simulink model "DP_STD_MDL_DCAC_3ph_2level_gridconn"  (R2024b)
settings: Solver=VariableStepAuto  StartTime=0.0  StopTime=6  RelTol=1e-3
libraries: spsSeriesRLCBranchLib x18, spsSecondOrderFilterLib x7, spsVoltageMeasurementLib x7, spsControlledVoltageSourceLib x4, spsMosfetLib x4, spsCurrentMeasurementLib x3, simulink x2, gmp_sil_core_pack x1, gmp_peripheral_utilities x1, spsdq0toabcLib x1, sps_lib x1
(part 2 of 2)

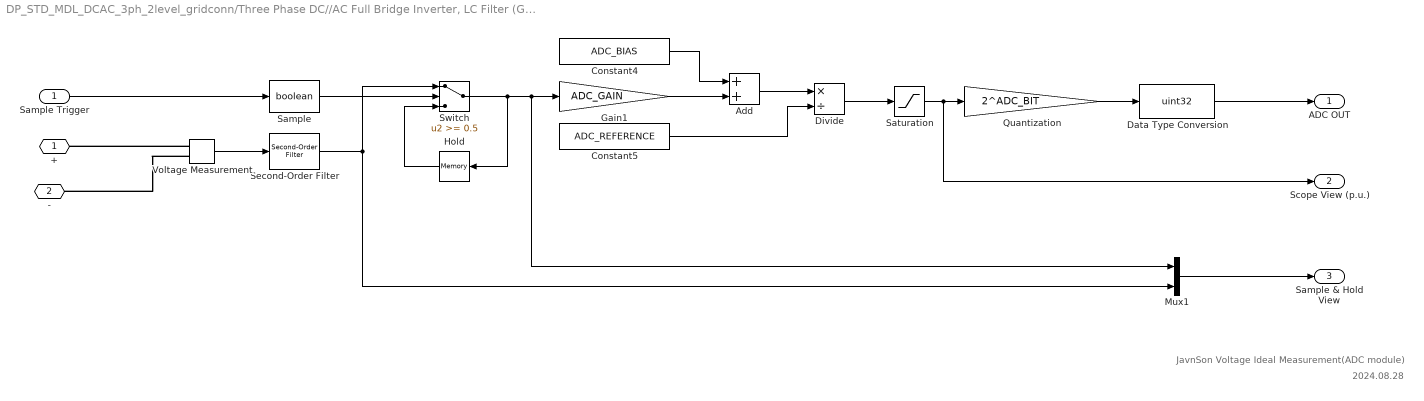
== system DP_STD_MDL_DCAC_3ph_2level_gridconn/Three Phase DC//AC Full Bridge Inverter, LC Filter (GMP STD MDL)/Capactor Voltage Uab Measurement Module1 ==
  note: 2024.08.28
  note: JavnSon Voltage Ideal Measurement(ADC module)
  Sample Trigger : Inport
  Add : Sum
  Constant4 : Constant  Value=ADC_BIAS
  Constant5 : Constant  Value=ADC_REFERENCE
  Data Type Conversion : DataTypeConversion  OutDataTypeStr=uint32  ConvertRealWorld=Stored Integer (SI)  SaturateOnIntegerOverflow=off  RndMeth=Floor
  Divide : Product  Inputs=*/
  Gain1 : Gain  Gain=ADC_GAIN
  Hold : Memory  InitialCondition=ADC_INIT  LinearizeAsDelay=on
  Mux1 : Mux  Inputs=2
  Quantization : Gain  Gain=2^ADC_BIT
  Sample : DataTypeConversion  OutDataTypeStr=boolean  SaturateOnIntegerOverflow=off  RndMeth=Floor
  Saturation : Saturate  UpperLimit=1  LowerLimit=0
  Second-Order Filter : spsSecondOrderFilterLib/Second-Order Filter  FilterType=Lowpass  Fo=cut_frequency  Zeta=0.707  Ts=0  Initialize=off  Vac_Init="[0,  0,  60]"  Vdc_Init=0  PlotResponse=off  FreqRange=[0, 500, 1]
  Switch : Switch  Threshold=0.5
  Voltage Measurement : spsVoltageMeasurementLib/Voltage Measurement  PhasorSimulation=off  OutputType=Complex  PSBequivalent=0
  + : PMIOPort  Side=Left
  - : PMIOPort  Port=2  Side=Left
  ADC OUT : Outport
  Scope View (p.u.) : Outport  Port=2
  Sample & Hold View : Outport  Port=3
  wires:
  Sample/1 -> Switch/2
  Add/1 -> Divide/1
  Constant5/1 -> Divide/2
  Quantization/1 -> Data Type Conversion/1
  Mux1/1 -> Sample & Hold View/1
  Data Type Conversion/1 -> ADC OUT/1
  Sample Trigger/1 -> Sample/1
  Gain1/1 -> Add/2
  Constant4/1 -> Add/1
  Saturation/1 -> Quantization/1, Scope View (p.u.)/1
  Voltage Measurement/1 -> Second-Order Filter/1
  Divide/1 -> Saturation/1
  Switch/1 -> Gain1/1, Mux1/1, Hold/1
  Hold/1 -> Switch/3
  Second-Order Filter/1 -> Switch/1, Mux1/2
  connections:
  Voltage Measurement/LConn2 -- -/RConn1
  Voltage Measurement/LConn1 -- +/RConn1

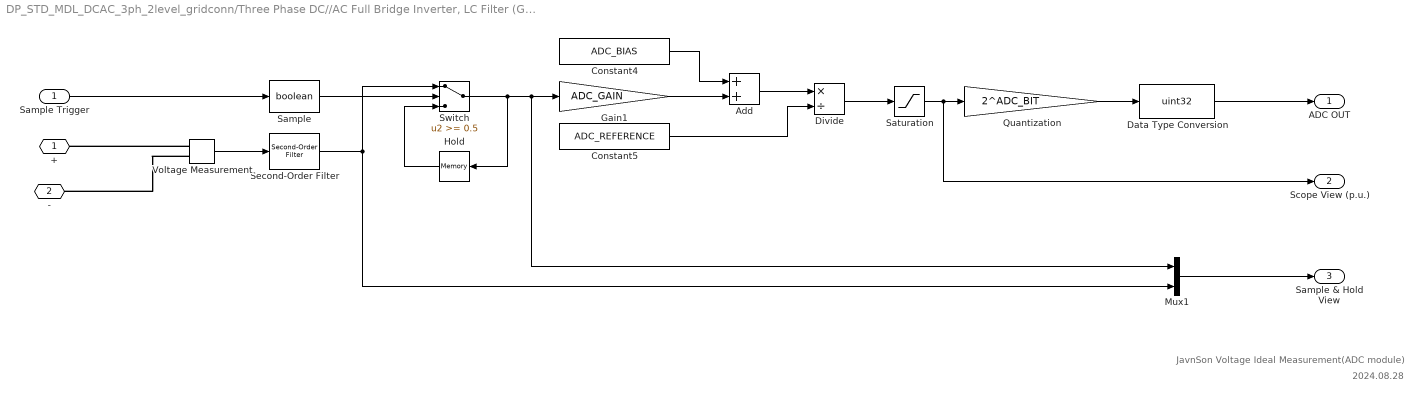
== system DP_STD_MDL_DCAC_3ph_2level_gridconn/Three Phase DC//AC Full Bridge Inverter, LC Filter (GMP STD MDL)/Capactor Voltage Ubc Measurement Module5 ==
  note: JavnSon Voltage Ideal Measurement(ADC module)
  note: 2024.08.28
  Sample Trigger : Inport
  Add : Sum
  Constant4 : Constant  Value=ADC_BIAS
  Constant5 : Constant  Value=ADC_REFERENCE
  Data Type Conversion : DataTypeConversion  OutDataTypeStr=uint32  ConvertRealWorld=Stored Integer (SI)  SaturateOnIntegerOverflow=off  RndMeth=Floor
  Divide : Product  Inputs=*/
  Gain1 : Gain  Gain=ADC_GAIN
  Hold : Memory  InitialCondition=ADC_INIT  LinearizeAsDelay=on
  Mux1 : Mux  Inputs=2
  Quantization : Gain  Gain=2^ADC_BIT
  Sample : DataTypeConversion  OutDataTypeStr=boolean  SaturateOnIntegerOverflow=off  RndMeth=Floor
  Saturation : Saturate  UpperLimit=1  LowerLimit=0
  Second-Order Filter : spsSecondOrderFilterLib/Second-Order Filter  FilterType=Lowpass  Fo=cut_frequency  Zeta=0.707  Ts=0  Initialize=off  Vac_Init="[0,  0,  60]"  Vdc_Init=0  PlotResponse=off  FreqRange=[0, 500, 1]
  Switch : Switch  Threshold=0.5
  Voltage Measurement : spsVoltageMeasurementLib/Voltage Measurement  PhasorSimulation=off  OutputType=Complex  PSBequivalent=0
  + : PMIOPort  Side=Left
  - : PMIOPort  Port=2  Side=Left
  ADC OUT : Outport
  Scope View (p.u.) : Outport  Port=2
  Sample & Hold View : Outport  Port=3
  wires:
  Second-Order Filter/1 -> Mux1/2, Switch/1
  Hold/1 -> Switch/3
  Switch/1 -> Hold/1, Mux1/1, Gain1/1
  Divide/1 -> Saturation/1
  Voltage Measurement/1 -> Second-Order Filter/1
  Saturation/1 -> Scope View (p.u.)/1, Quantization/1
  Constant4/1 -> Add/1
  Gain1/1 -> Add/2
  Sample Trigger/1 -> Sample/1
  Data Type Conversion/1 -> ADC OUT/1
  Mux1/1 -> Sample & Hold View/1
  Quantization/1 -> Data Type Conversion/1
  Constant5/1 -> Divide/2
  Add/1 -> Divide/1
  Sample/1 -> Switch/2
  connections:
  Voltage Measurement/LConn1 -- +/RConn1
  Voltage Measurement/LConn2 -- -/RConn1

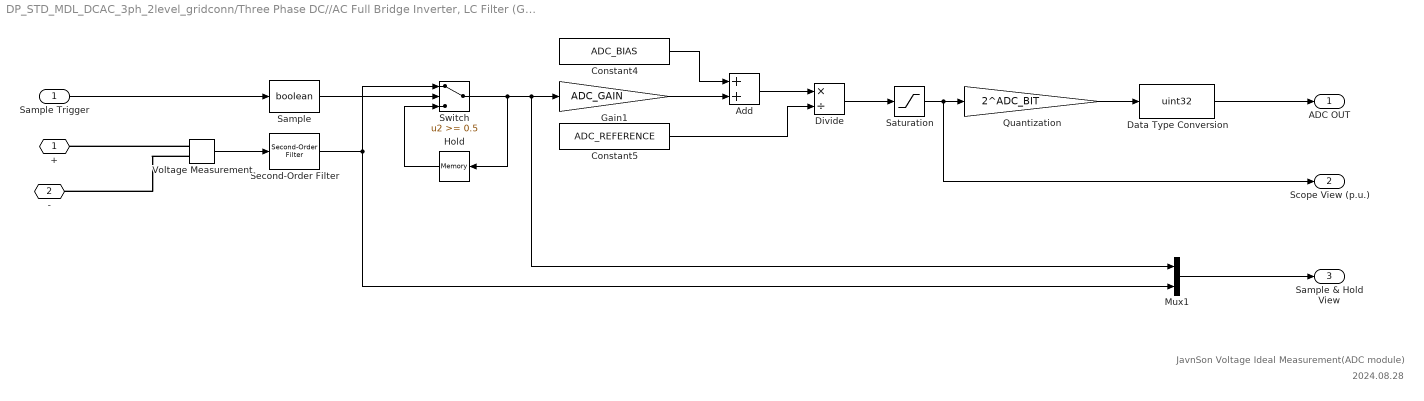
== system DP_STD_MDL_DCAC_3ph_2level_gridconn/Three Phase DC//AC Full Bridge Inverter, LC Filter (GMP STD MDL)/DC Bus Current Measurement Module ==
  note: 2024.08.28
  note: JavnSon Voltage Ideal Measurement(ADC module)
  Sample Trigger : Inport
  Add : Sum
  Constant4 : Constant  Value=ADC_BIAS
  Constant5 : Constant  Value=ADC_REFERENCE
  Data Type Conversion : DataTypeConversion  OutDataTypeStr=uint32  ConvertRealWorld=Stored Integer (SI)  SaturateOnIntegerOverflow=off  RndMeth=Floor
  Divide : Product  Inputs=*/
  Gain1 : Gain  Gain=ADC_GAIN
  Hold : Memory  InitialCondition=ADC_INIT  LinearizeAsDelay=on
  Mux1 : Mux  Inputs=2
  Quantization : Gain  Gain=2^ADC_BIT
  Sample : DataTypeConversion  OutDataTypeStr=boolean  SaturateOnIntegerOverflow=off  RndMeth=Floor
  Saturation : Saturate  UpperLimit=1  LowerLimit=0
  Second-Order Filter : spsSecondOrderFilterLib/Second-Order Filter  FilterType=Lowpass  Fo=cut_frequency  Zeta=0.707  Ts=0  Initialize=off  Vac_Init="[0,  0,  60]"  Vdc_Init=0  PlotResponse=off  FreqRange=[0, 500, 1]
  Switch : Switch  Threshold=0.5
  Voltage Measurement : spsVoltageMeasurementLib/Voltage Measurement  PhasorSimulation=off  OutputType=Complex  PSBequivalent=0
  + : PMIOPort  Side=Left
  - : PMIOPort  Port=2  Side=Left
  ADC OUT : Outport
  Scope View (p.u.) : Outport  Port=2
  Sample & Hold View : Outport  Port=3
  wires:
  Sample/1 -> Switch/2
  Add/1 -> Divide/1
  Constant5/1 -> Divide/2
  Quantization/1 -> Data Type Conversion/1
  Mux1/1 -> Sample & Hold View/1
  Data Type Conversion/1 -> ADC OUT/1
  Sample Trigger/1 -> Sample/1
  Gain1/1 -> Add/2
  Constant4/1 -> Add/1
  Saturation/1 -> Quantization/1, Scope View (p.u.)/1
  Voltage Measurement/1 -> Second-Order Filter/1
  Divide/1 -> Saturation/1
  Switch/1 -> Gain1/1, Mux1/1, Hold/1
  Hold/1 -> Switch/3
  Second-Order Filter/1 -> Switch/1, Mux1/2
  connections:
  Voltage Measurement/LConn2 -- -/RConn1
  Voltage Measurement/LConn1 -- +/RConn1

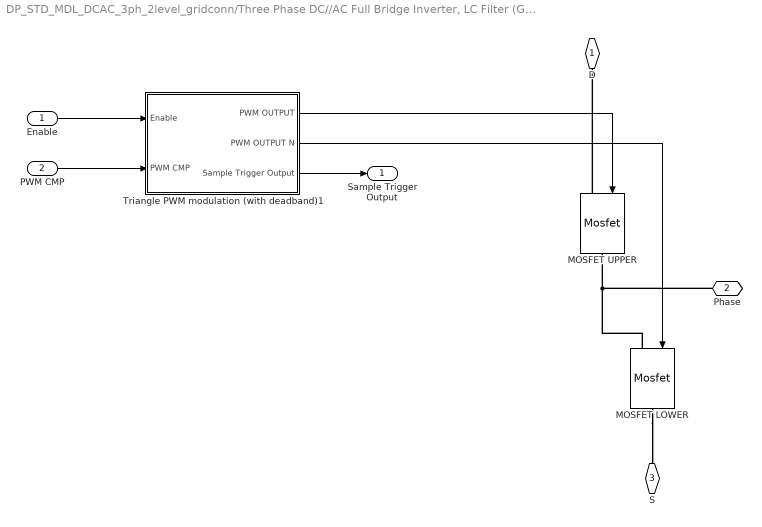
== system DP_STD_MDL_DCAC_3ph_2level_gridconn/Three Phase DC//AC Full Bridge Inverter, LC Filter (GMP STD MDL)/Single Phase Full Bridge (Duty Model) phase U ==
  Enable : Inport
  PWM CMP : Inport  Port=2
  MOSFET LOWER : spsMosfetLib/Mosfet  Ron=R_mosfet_on  Lon=Lon  Rd=Rd  Vfd=Vf  IC=0  Rs=Rs  Cs=Cs  Measurements=off
  MOSFET UPPER : spsMosfetLib/Mosfet  Ron=R_mosfet_on  Lon=Lon  Rd=Rd  Vfd=Vf  IC=0  Rs=Rs  Cs=Cs  Measurements=off
  Triangle PWM modulation (with deadband)1 : Subsystem  mask{fswitch=fswitch, CMP_MAX=CMP_MAX, Deadband_Upper=Deadband_Upper, Deadband_Lower=Deadband_Lower, Deadband_us=NaN, phase_shift=phase_shift}
      mask prompts: Deadband_us "Deadband Time: (μs)"
      mask init:
      | calculate_deadband(gcb, 'Deadband_Upper', 'Deadband_Lower',	'CMP_MAX', 'fswitch', 'Deadband_us');
      mask Callback fswitch: calculate_deadband(gcb, 'Deadband_Upper', 'Deadband_Lower',	'CMP_MAX', 'fswitch', 'Deadband_us');
      mask Callback CMP_MAX: calculate_deadband(gcb, 'Deadband_Upper', 'Deadband_Lower',	'CMP_MAX', 'fswitch', 'Deadband_us');
      mask Callback Deadband_Upper:
      | calculate_deadband(gcb, 'Deadband_Upper', 'Deadband_Lower',	'CMP_MAX', 'fswitch', 'Deadband_us');
      | 
      | % Get handle of Mask
      | %mask_obj = Simulink.Mask.get(gcb);
      | %Parameters = Simulink.Mask.get(gcb).Parameters;
      | 
      | % Get source data
      | %dead_band_up = str2double(Parameters(strcmp(get_param(gcb,'MaskNames'),'Deadband_Upper')==1).Value);
      | %dead_band_dn = str2double(Parameters(strcmp(get_param(gcb,'MaskNames'),'Deadband_Lower')==1).Value);
      | %cmp_max = str2double(Parameters(strcmp(get_param(gcb,'MaskNames'),'CMP_MAX')==1).Value);
      | %switch_freq = str2double(Parameters(strcmp(get_param(gcb,'MaskNames'),'fswitch')==1).Value);
      | 
      | % calculate deadband
      | %dead_band_us = 1/switch_freq * (dead_band_up + dead_band_dn) / cmp_max*1e6;
      | 
      | % Set result
      | %Parameters(strcmp(get_param(gcb,'MaskNames'),'Deadband_upper_us')==1).Value=num2str(dead_band_us);
      mask Callback Deadband_Lower: calculate_deadband(gcb, 'Deadband_Upper', 'Deadband_Lower',	'CMP_MAX', 'fswitch', 'Deadband_upper_us');
      mask DialogControl DescGroupVar Prompt: PWM Modulator
      mask DialogControl Control8 Prompt: GMP CTL Simulink Utilities: virtual peripherals
      mask DialogControl DescTextVar Prompt: PWM Modulator. Input PWM compare register value, output ADC trigger signal, PWM output and negtive PWM output.
      mask DialogControl ParameterGroupVar Prompt: 参数
      mask DialogControl Control2 Prompt: PWM Frequency (Hz) :
      mask DialogControl Control4 Prompt: Full Scale PWM Compare value:
      mask DialogControl Control5 Prompt: (whole period is 2 * CMP_MAX ticks)
      mask DialogControl Control3 Prompt: Deadband Range Set (CMP Value):
      mask DialogControl Control6 Prompt: Single side deadband time: DEADBAND_CMP/2/CMP_MAX/fswitch
      mask DialogControl Control7 Prompt: Initial Phase (rad)
  D : PMIOPort  Side=Left
  Phase : PMIOPort  Port=2  Side=Right
  S : PMIOPort  Port=3  Side=Right
  Sample Trigger Output : Outport
  wires:
  Triangle PWM modulation (with deadband)1/1(PWM OUTPUT) -> MOSFET UPPER/1
  Enable/1 -> Triangle PWM modulation (with deadband)1/1(Enable)
  Triangle PWM modulation (with deadband)1/3(Sample Trigger Output) -> Sample Trigger Output/1
  Triangle PWM modulation (with deadband)1/2(PWM OUTPUT N) -> MOSFET LOWER/1
  PWM CMP/1 -> Triangle PWM modulation (with deadband)1/2(PWM CMP)
  connections:
  MOSFET UPPER/LConn1 -- D/RConn1
  MOSFET LOWER/LConn1 -- Phase/RConn1 -- MOSFET UPPER/RConn1
  MOSFET LOWER/RConn1 -- S/RConn1

== system DP_STD_MDL_DCAC_3ph_2level_gridconn/Three Phase DC//AC Full Bridge Inverter, LC Filter (GMP STD MDL)/Single Phase Full Bridge (Duty Model) phase V ==
  Enable : Inport
  PWM CMP : Inport  Port=2
  MOSFET LOWER : spsMosfetLib/Mosfet  Ron=R_mosfet_on  Lon=Lon  Rd=Rd  Vfd=Vf  IC=0  Rs=Rs  Cs=Cs  Measurements=off
  MOSFET UPPER : spsMosfetLib/Mosfet  Ron=R_mosfet_on  Lon=Lon  Rd=Rd  Vfd=Vf  IC=0  Rs=Rs  Cs=Cs  Measurements=off
  Triangle PWM modulation (with deadband)1 : Subsystem  mask{fswitch=fswitch, CMP_MAX=CMP_MAX, Deadband_Upper=Deadband_Upper, Deadband_Lower=Deadband_Lower, Deadband_us=NaN, phase_shift=phase_shift}
      mask prompts: Deadband_us "Deadband Time: (μs)"
      mask init:
      | calculate_deadband(gcb, 'Deadband_Upper', 'Deadband_Lower',	'CMP_MAX', 'fswitch', 'Deadband_us');
      mask Callback fswitch: calculate_deadband(gcb, 'Deadband_Upper', 'Deadband_Lower',	'CMP_MAX', 'fswitch', 'Deadband_us');
      mask Callback CMP_MAX: calculate_deadband(gcb, 'Deadband_Upper', 'Deadband_Lower',	'CMP_MAX', 'fswitch', 'Deadband_us');
      mask Callback Deadband_Upper:
      | calculate_deadband(gcb, 'Deadband_Upper', 'Deadband_Lower',	'CMP_MAX', 'fswitch', 'Deadband_us');
      | 
      | % Get handle of Mask
      | %mask_obj = Simulink.Mask.get(gcb);
      | %Parameters = Simulink.Mask.get(gcb).Parameters;
      | 
      | % Get source data
      | %dead_band_up = str2double(Parameters(strcmp(get_param(gcb,'MaskNames'),'Deadband_Upper')==1).Value);
      | %dead_band_dn = str2double(Parameters(strcmp(get_param(gcb,'MaskNames'),'Deadband_Lower')==1).Value);
      | %cmp_max = str2double(Parameters(strcmp(get_param(gcb,'MaskNames'),'CMP_MAX')==1).Value);
      | %switch_freq = str2double(Parameters(strcmp(get_param(gcb,'MaskNames'),'fswitch')==1).Value);
      | 
      | % calculate deadband
      | %dead_band_us = 1/switch_freq * (dead_band_up + dead_band_dn) / cmp_max*1e6;
      | 
      | % Set result
      | %Parameters(strcmp(get_param(gcb,'MaskNames'),'Deadband_upper_us')==1).Value=num2str(dead_band_us);
      mask Callback Deadband_Lower: calculate_deadband(gcb, 'Deadband_Upper', 'Deadband_Lower',	'CMP_MAX', 'fswitch', 'Deadband_upper_us');
      mask DialogControl DescGroupVar Prompt: PWM Modulator
      mask DialogControl Control8 Prompt: GMP CTL Simulink Utilities: virtual peripherals
      mask DialogControl DescTextVar Prompt: PWM Modulator. Input PWM compare register value, output ADC trigger signal, PWM output and negtive PWM output.
      mask DialogControl ParameterGroupVar Prompt: 参数
      mask DialogControl Control2 Prompt: PWM Frequency (Hz) :
      mask DialogControl Control4 Prompt: Full Scale PWM Compare value:
      mask DialogControl Control5 Prompt: (whole period is 2 * CMP_MAX ticks)
      mask DialogControl Control3 Prompt: Deadband Range Set (CMP Value):
      mask DialogControl Control6 Prompt: Single side deadband time: DEADBAND_CMP/2/CMP_MAX/fswitch
      mask DialogControl Control7 Prompt: Initial Phase (rad)
  D : PMIOPort  Side=Left
  Phase : PMIOPort  Port=2  Side=Right
  S : PMIOPort  Port=3  Side=Right
  Sample Trigger Output : Outport
  wires:
  PWM CMP/1 -> Triangle PWM modulation (with deadband)1/2(PWM CMP)
  Triangle PWM modulation (with deadband)1/2(PWM OUTPUT N) -> MOSFET LOWER/1
  Triangle PWM modulation (with deadband)1/3(Sample Trigger Output) -> Sample Trigger Output/1
  Enable/1 -> Triangle PWM modulation (with deadband)1/1(Enable)
  Triangle PWM modulation (with deadband)1/1(PWM OUTPUT) -> MOSFET UPPER/1
  connections:
  MOSFET LOWER/RConn1 -- S/RConn1
  MOSFET UPPER/RConn1 -- Phase/RConn1 -- MOSFET LOWER/LConn1
  MOSFET UPPER/LConn1 -- D/RConn1

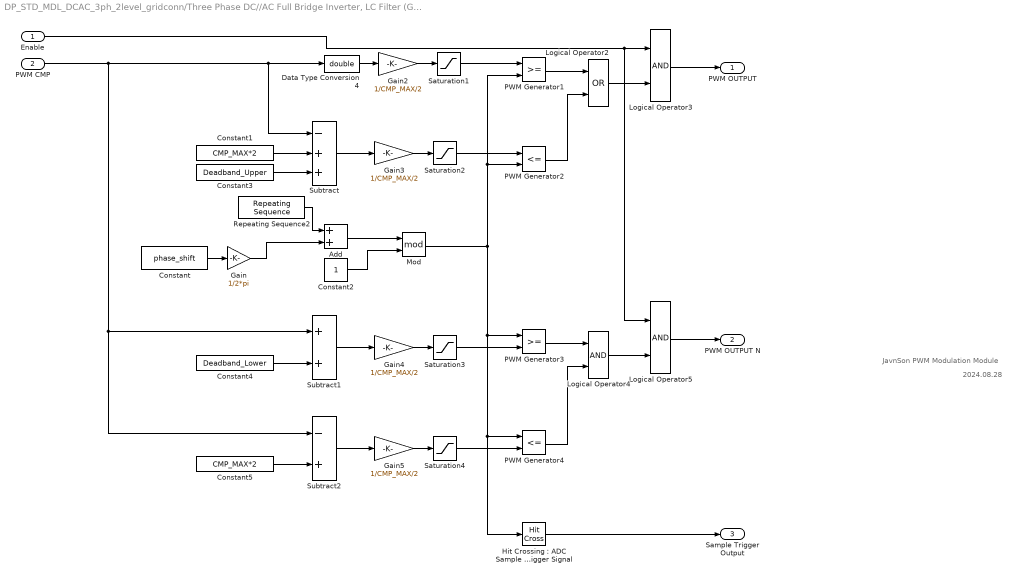
== system DP_STD_MDL_DCAC_3ph_2level_gridconn/Three Phase DC//AC Full Bridge Inverter, LC Filter (GMP STD MDL)/Single Phase Full Bridge (Duty Model) phase U/Triangle PWM modulation (with deadband)1 ==
  note: JavnSon PWM Modulation Module
  note: 2024.08.28
  Enable : Inport
  PWM CMP : Inport  Port=2
  Add : Sum
  Constant : Constant  Value=phase_shift
  Constant1 : Constant  Value=CMP_MAX*2
  Constant2 : Constant
  Constant3 : Constant  Value=Deadband_Upper
  Constant4 : Constant  Value=Deadband_Lower
  Constant5 : Constant  Value=CMP_MAX*2
  Data Type Conversion4 : DataTypeConversion  OutDataTypeStr=double  SaturateOnIntegerOverflow=off  RndMeth=Floor
  Gain : Gain  Gain=1/2*pi
  Gain{2..5} (4 alike) : Gain  Gain=1/CMP_MAX/2
  Hit Crossing：ADC Sample Trigger Signal : HitCross  HitCrossingOffset=0.5  HitCrossingDirection=rising
  Logical Operator2 : Logic  Operator=OR  AllPortsSameDT=off  OutDataTypeStr=boolean
  Logical Operator3 : Logic  AllPortsSameDT=off  OutDataTypeStr=boolean
  Logical Operator4 : Logic  AllPortsSameDT=off  OutDataTypeStr=boolean
  Logical Operator5 : Logic  AllPortsSameDT=off  OutDataTypeStr=boolean
  Mod : Math  Operator=mod
  PWM Generator1 : RelationalOperator  OutDataTypeStr=boolean  InputSameDT=off
  PWM Generator2 : RelationalOperator  Operator=<=  OutDataTypeStr=boolean  InputSameDT=off
  PWM Generator3 : RelationalOperator  OutDataTypeStr=boolean  InputSameDT=off
  PWM Generator4 : RelationalOperator  Operator=<=  OutDataTypeStr=boolean  InputSameDT=off
  Repeating Sequence2 : simulink/Sources/Repeating Sequence  rep_seq_t=[0, 1/2/fswitch, 1/fswitch ]  rep_seq_y=[0,0.5,1]
  Saturation{1..4} (4 alike) : Saturate  UpperLimit=1  LowerLimit=0
  Subtract : Sum  Inputs=-++
  Subtract1 : Sum
  Subtract2 : Sum  Inputs=-+
  PWM OUTPUT : Outport
  PWM OUTPUT N : Outport  Port=2
  Sample Trigger Output : Outport  Port=3
  wires:
  Constant/1 -> Gain/1
  Constant2/1 -> Mod/2
  Add/1 -> Mod/1
  Gain/1 -> Add/2
  Repeating Sequence2/1 -> Add/1
  Hit Crossing：ADC Sample Trigger Signal/1 -> Sample Trigger Output/1
  Logical Operator3/1 -> PWM OUTPUT/1
  Logical Operator5/1 -> PWM OUTPUT N/1
  Enable/1 -> Logical Operator3/1, Logical Operator5/1
  Mod/1 -> PWM Generator4/1, Hit Crossing：ADC Sample Trigger Signal/1, PWM Generator3/1, PWM Generator1/2, PWM Generator2/2
  Logical Operator4/1 -> Logical Operator5/2
  PWM Generator4/1 -> Logical Operator4/2
  Subtract2/1 -> Gain5/1
  Gain5/1 -> Saturation4/1
  Saturation4/1 -> PWM Generator4/2
  Constant5/1 -> Subtract2/2
  PWM Generator3/1 -> Logical Operator4/1
  Saturation3/1 -> PWM Generator3/2
  Subtract1/1 -> Gain4/1
  Gain4/1 -> Saturation3/1
  Constant4/1 -> Subtract1/2
  Saturation2/1 -> PWM Generator2/1
  Subtract/1 -> Gain3/1
  Gain3/1 -> Saturation2/1
  PWM Generator2/1 -> Logical Operator2/2
  Constant3/1 -> Subtract/3
  Constant1/1 -> Subtract/2
  Logical Operator2/1 -> Logical Operator3/2
  PWM Generator1/1 -> Logical Operator2/1
  Saturation1/1 -> PWM Generator1/1
  Gain2/1 -> Saturation1/1
  Data Type Conversion4/1 -> Gain2/1
  PWM CMP/1 -> Data Type Conversion4/1, Subtract/1, Subtract1/1, Subtract2/1

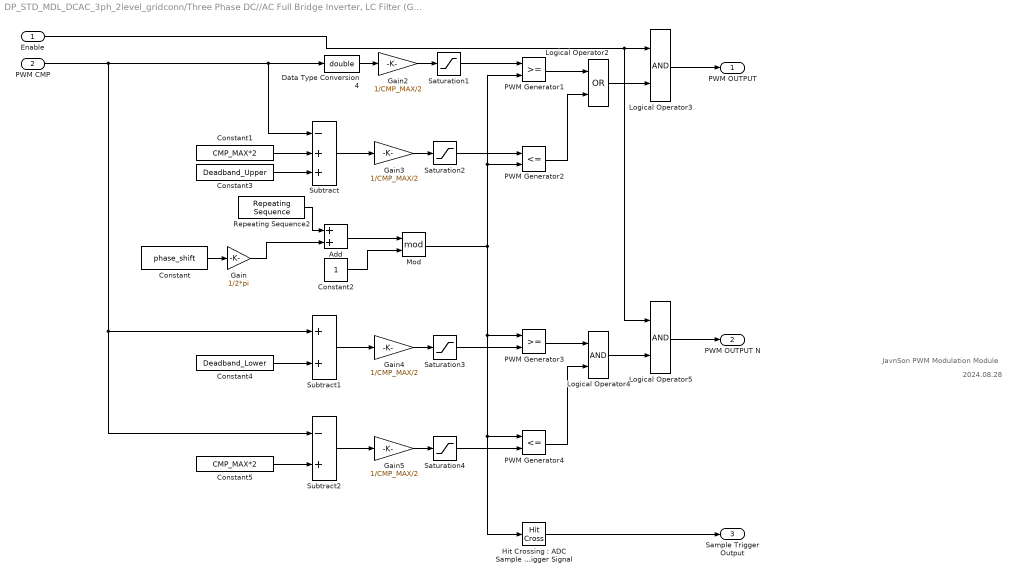
== system DP_STD_MDL_DCAC_3ph_2level_gridconn/Three Phase DC//AC Full Bridge Inverter, LC Filter (GMP STD MDL)/Single Phase Full Bridge (Duty Model) phase V/Triangle PWM modulation (with deadband)1 ==
  note: 2024.08.28
  note: JavnSon PWM Modulation Module
  Enable : Inport
  PWM CMP : Inport  Port=2
  Add : Sum
  Constant : Constant  Value=phase_shift
  Constant1 : Constant  Value=CMP_MAX*2
  Constant2 : Constant
  Constant3 : Constant  Value=Deadband_Upper
  Constant4 : Constant  Value=Deadband_Lower
  Constant5 : Constant  Value=CMP_MAX*2
  Data Type Conversion4 : DataTypeConversion  OutDataTypeStr=double  SaturateOnIntegerOverflow=off  RndMeth=Floor
  Gain : Gain  Gain=1/2*pi
  Gain{2..5} (4 alike) : Gain  Gain=1/CMP_MAX/2
  Hit Crossing：ADC Sample Trigger Signal : HitCross  HitCrossingOffset=0.5  HitCrossingDirection=rising
  Logical Operator2 : Logic  Operator=OR  AllPortsSameDT=off  OutDataTypeStr=boolean
  Logical Operator3 : Logic  AllPortsSameDT=off  OutDataTypeStr=boolean
  Logical Operator4 : Logic  AllPortsSameDT=off  OutDataTypeStr=boolean
  Logical Operator5 : Logic  AllPortsSameDT=off  OutDataTypeStr=boolean
  Mod : Math  Operator=mod
  PWM Generator1 : RelationalOperator  OutDataTypeStr=boolean  InputSameDT=off
  PWM Generator2 : RelationalOperator  Operator=<=  OutDataTypeStr=boolean  InputSameDT=off
  PWM Generator3 : RelationalOperator  OutDataTypeStr=boolean  InputSameDT=off
  PWM Generator4 : RelationalOperator  Operator=<=  OutDataTypeStr=boolean  InputSameDT=off
  Repeating Sequence2 : simulink/Sources/Repeating Sequence  rep_seq_t=[0, 1/2/fswitch, 1/fswitch ]  rep_seq_y=[0,0.5,1]
  Saturation{1..4} (4 alike) : Saturate  UpperLimit=1  LowerLimit=0
  Subtract : Sum  Inputs=-++
  Subtract1 : Sum
  Subtract2 : Sum  Inputs=-+
  PWM OUTPUT : Outport
  PWM OUTPUT N : Outport  Port=2
  Sample Trigger Output : Outport  Port=3
  wires:
  PWM CMP/1 -> Subtract2/1, Subtract1/1, Subtract/1, Data Type Conversion4/1
  Data Type Conversion4/1 -> Gain2/1
  Gain2/1 -> Saturation1/1
  Saturation1/1 -> PWM Generator1/1
  PWM Generator1/1 -> Logical Operator2/1
  Logical Operator2/1 -> Logical Operator3/2
  Constant1/1 -> Subtract/2
  Constant3/1 -> Subtract/3
  PWM Generator2/1 -> Logical Operator2/2
  Gain3/1 -> Saturation2/1
  Subtract/1 -> Gain3/1
  Saturation2/1 -> PWM Generator2/1
  Constant4/1 -> Subtract1/2
  Gain4/1 -> Saturation3/1
  Subtract1/1 -> Gain4/1
  Saturation3/1 -> PWM Generator3/2
  PWM Generator3/1 -> Logical Operator4/1
  Constant5/1 -> Subtract2/2
  Saturation4/1 -> PWM Generator4/2
  Gain5/1 -> Saturation4/1
  Subtract2/1 -> Gain5/1
  PWM Generator4/1 -> Logical Operator4/2
  Logical Operator4/1 -> Logical Operator5/2
  Mod/1 -> PWM Generator2/2, PWM Generator1/2, PWM Generator3/1, Hit Crossing：ADC Sample Trigger Signal/1, PWM Generator4/1
  Enable/1 -> Logical Operator5/1, Logical Operator3/1
  Logical Operator5/1 -> PWM OUTPUT N/1
  Logical Operator3/1 -> PWM OUTPUT/1
  Hit Crossing：ADC Sample Trigger Signal/1 -> Sample Trigger Output/1
  Repeating Sequence2/1 -> Add/1
  Gain/1 -> Add/2
  Add/1 -> Mod/1
  Constant2/1 -> Mod/2
  Constant/1 -> Gain/1
